simulink model "test_semiconductors_bridges"  (R2026b)
settings: Solver=ode23tb  StopTime=tb.t_stop
undefined symbols (not defined in the file or in its folder): tb
libraries: fl_lib x144, nesl_utility x54, single_phase_pwm_modulator x1, full_bridge_two_level_ideal_switch x1, full_bridge_two_level_igbt_simple_2th x1, full_bridge_two_level_mos_simple_2th x1, single_phase_three_levels_PWM_modulator x1, full_bridge_three_level_ttype_ideal_switch x1, full_bridge_three_level_ttype_igbt_simple_2th x1, full_bridge_three_level_ttype_mos_simple_2th x1, half_bridge_three_level_ttype_ideal_switch x1, half_bridge_three_level_ttype_igbt_simple_2th x1
(part 2 of 3)

== system test_semiconductors_bridges/modulator_1ph3L/test_half_bridge_three_level_ttype_mos_simple_2th ==
  gate_commands : Inport
  Electrical Reference : fl_lib/Electrical/Electrical Elements/Electrical Reference
  L : fl_lib/Electrical/Electrical Elements/Inductor  l=tb.load.L H  r=0 Ohm  g=0 1/Ohm  i_specify=off  i_priority=None  i=0 A  i_nominal_specify=off  i_nominal_value=1  i_nominal_unit=A  v_specify=off  v_priority=None  v=0 V  v_nominal_specify=off  v_nominal_value=1  v_nominal_unit=V  i_L_specify=off  i_L_priority=High  i_L=0 A  i_L_nominal_specify=off  i_L_nominal_value=1  i_L_nominal_unit=A
  R : fl_lib/Electrical/Electrical Elements/Resistor  R=tb.load.R Ohm  i_specify=off  i_priority=None  i=0 A  i_nominal_specify=off  i_nominal_value=1  i_nominal_unit=A  v_specify=off  v_priority=None  v=0 V  v_nominal_specify=off  v_nominal_value=1  v_nominal_unit=V
  Solver Configuration : nesl_utility/Solver Configuration  PhysicalDomain=network_engine_domain  SubClassName=solver  LeftPortType=input  RightPortType=generic  Tones=[]  Harmonics=[]  SimulateNoise=off  Profile=off  UseLocalSampling=off  EnableSwitchedLinearOptims=on  FrequencyDomain=off  UseCCode=off  RelTol=0.001  AbsTol=0.001  MinStep=1e-09  ToWorkspace=off  RevertToSquareIcSolve=off  NumHomotopyIterations=100  PhasorMode=off  PhasorModeNumHarmonics=1  ConsistencySolver=NEWTON_FTOL  CanonicalOrdering=UNORDERED  OptimizeIntermediates=UNOPTIMIZED  MulticoreSolverChoice=BACKWARD_EULER  IndexReductionMethod=DerivativeReplacement  DoDC=off  ResidualTolerance=1e-4  ConsistencyTolSource=GLOBAL  ConsistencyAbsTol=0.001  ConsistencyRelTol=0.001  ConsistencyTolFactor=0.001  UseLocalSolver=on  LocalSolverChoice=NE_BACKWARD_EULER_ADVANCER  ResolveIndetEquations=on  FunctionEvalNumThread=1  LocalSolverSampleTime=tb.tc  DoFixedCost=on  MaxNonlinIter=tb.nonlin_iter_ttype  MaxModeIter=tb.mode_iter  ComputeImpulses=off  ImpulseIterations=2  LinearAlgebra=auto  LinearAlgebraNumThread=0  EquationFormulation=NE_TIME_EF  DelaysMemoryBudget=1024  AutomaticFiltering=on  FilteringTimeConstant=0.001  PartitionStorageMethod=AS_NEEDED  PartitionMemoryBudget=1024  PartitionMethod=BALANCED  MultibodyUseLocalSolver=off  MultibodyLocalSolverChoice=ODE1  MultibodyLocalSolverSampleTime=0.001
  Vdc1 : fl_lib/Electrical/Electrical Sources/DC Voltage Source  v0=tb.Vdc/2 V
  Vdc2 : fl_lib/Electrical/Electrical Sources/DC Voltage Source  v0=tb.Vdc/2 V
  half_bridge_three_level_ttype_mos_simple_2th : half_bridge_three_level_ttype_mos_simple_2th/half_bridge_three_level_ttype_mos_simple_2th  rds_on_m=tb.mos.rds_on  alpha_R_m=tb.mos.alpha_R  Tj_ref_m=tb.mos.Tj_ref  Roff_m=tb.mos.Roff  v_gamma_m=tb.mos.v_gamma  rd_on_m=tb.mos.rd_on  two_die_m=tb.mos.two_die  G_th_m=tb.mos.G_th  Eon_m=tb.mos.Eon  Eoff_m=tb.mos.Eoff  Err_m=tb.mos.Err  Ic_ref_m=tb.mos.Ic_ref  Vdc_ref_m=tb.mos.Vdc_ref  ki_m=tb.mos.ki  kv_m=tb.mos.kv  Vth_off_m=tb.mos.Vth_off  Vth_on_m=tb.mos.Vth_on  V_sm_m=tb.mos.V_sm  time_constant_edge_m=tb.mos.time_constant_edge  tau_v_m=tb.mos.tau_v  time_constant_ploss_m=tb.mos.time_constant_ploss  i_eps_m=tb.mos.i_eps  Csnubber_m=tb.mos.Csnubber  Rsnubber_m=tb.mos.Rsnubber  rth_switch_JH_m=tb.mos.rth_switch_JH  rth_switch_HA_m=tb.mos.rth_switch_HA  rth_diode_JH_m=tb.mos.rth_diode_JH  rth_diode_HA_m=tb.mos.rth_diode_HA  JunctionTermalMass_m=tb.mos.JunctionTermalMass  Tambient_m=tb.mos.Tambient  mass_heatsink_m=tb.mos.mass_heatsink  specific_heat_m=tb.mos.specific_heat
  half_bridge_three_level_ttype_mos_simple_2th_i : ToWorkspace  VariableName=half_bridge_three_level_ttype_mos_simple_2th_i  SaveFormat=Timeseries  SampleTime=tb.ts_log
  half_bridge_three_level_ttype_mos_simple_2th_m : ToWorkspace  VariableName=half_bridge_three_level_ttype_mos_simple_2th_m  SaveFormat=Timeseries  SampleTime=tb.ts_log
  half_bridge_three_level_ttype_mos_simple_2th_u : ToWorkspace  VariableName=half_bridge_three_level_ttype_mos_simple_2th_u  SaveFormat=Timeseries  SampleTime=tb.ts_log
  i_A : nesl_utility/PS-Simulink Converter  PhysicalDomain=network_engine_domain  SubClassName=ps_output  LeftPortType=input  RightPortType=output  PseudoPeriodic=off  Frequencies=[]  VectorFormat=1-D array  Unit=A  AffineConversion=off
  i_load : fl_lib/Electrical/Electrical Sensors/Current Sensor
  u_V : nesl_utility/PS-Simulink Converter  PhysicalDomain=network_engine_domain  SubClassName=ps_output  LeftPortType=input  RightPortType=output  PseudoPeriodic=off  Frequencies=[]  VectorFormat=1-D array  Unit=V  AffineConversion=off
  u_load : fl_lib/Electrical/Electrical Sensors/Voltage Sensor
  wires:
  gate_commands/1 -> half_bridge_three_level_ttype_mos_simple_2th/1
  half_bridge_three_level_ttype_mos_simple_2th/1 -> half_bridge_three_level_ttype_mos_simple_2th_m/1
  i_A/1 -> half_bridge_three_level_ttype_mos_simple_2th_i/1
  u_V/1 -> half_bridge_three_level_ttype_mos_simple_2th_u/1
  connections:
  Vdc1/LConn1 -- half_bridge_three_level_ttype_mos_simple_2th/LConn1
  Vdc2/RConn1 -- half_bridge_three_level_ttype_mos_simple_2th/LConn3
  i_load/RConn1 -- i_A/LConn1
  u_load/RConn1 -- u_V/LConn1
  half_bridge_three_level_ttype_mos_simple_2th/RConn1 -- i_load/LConn1 -- u_load/LConn1
  i_load/RConn2 -- R/LConn1
  R/RConn1 -- L/LConn1
  L/RConn1 -- u_load/RConn2 -- Vdc1/RConn1 -- Vdc2/LConn1 -- Electrical Reference/LConn1 -- Solver Configuration/RConn1 -- half_bridge_three_level_ttype_mos_simple_2th/LConn2

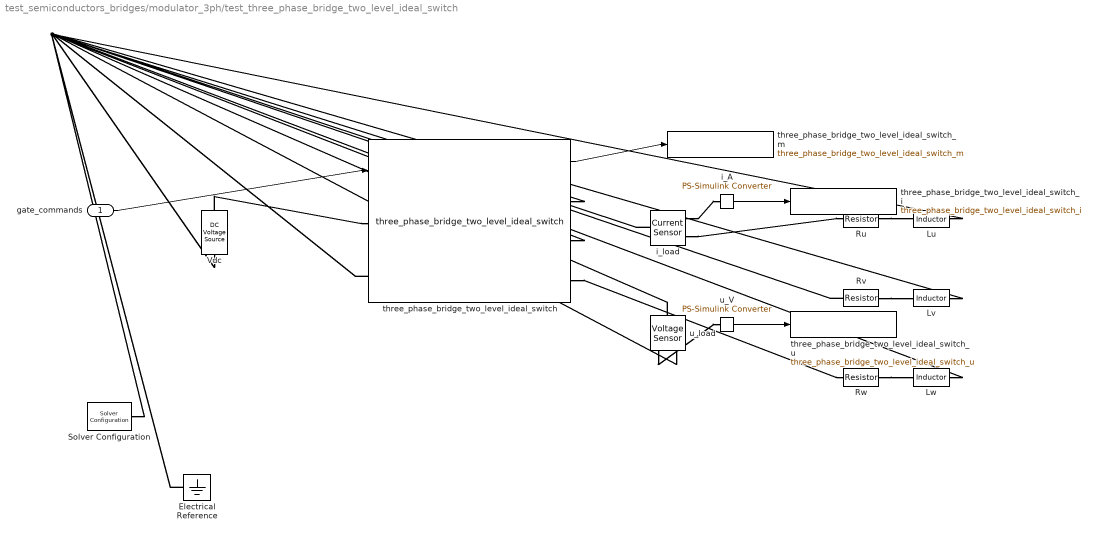
== system test_semiconductors_bridges/modulator_3ph/test_three_phase_bridge_two_level_ideal_switch ==
  gate_commands : Inport
  Electrical Reference : fl_lib/Electrical/Electrical Elements/Electrical Reference
  Lu : fl_lib/Electrical/Electrical Elements/Inductor  l=tb.load.L H  r=0 Ohm  g=0 1/Ohm  i_specify=off  i_priority=None  i=0 A  i_nominal_specify=off  i_nominal_value=1  i_nominal_unit=A  v_specify=off  v_priority=None  v=0 V  v_nominal_specify=off  v_nominal_value=1  v_nominal_unit=V  i_L_specify=off  i_L_priority=High  i_L=0 A  i_L_nominal_specify=off  i_L_nominal_value=1  i_L_nominal_unit=A
  Lv : fl_lib/Electrical/Electrical Elements/Inductor  l=tb.load.L H  r=0 Ohm  g=0 1/Ohm  i_specify=off  i_priority=None  i=0 A  i_nominal_specify=off  i_nominal_value=1  i_nominal_unit=A  v_specify=off  v_priority=None  v=0 V  v_nominal_specify=off  v_nominal_value=1  v_nominal_unit=V  i_L_specify=off  i_L_priority=High  i_L=0 A  i_L_nominal_specify=off  i_L_nominal_value=1  i_L_nominal_unit=A
  Lw : fl_lib/Electrical/Electrical Elements/Inductor  l=tb.load.L H  r=0 Ohm  g=0 1/Ohm  i_specify=off  i_priority=None  i=0 A  i_nominal_specify=off  i_nominal_value=1  i_nominal_unit=A  v_specify=off  v_priority=None  v=0 V  v_nominal_specify=off  v_nominal_value=1  v_nominal_unit=V  i_L_specify=off  i_L_priority=High  i_L=0 A  i_L_nominal_specify=off  i_L_nominal_value=1  i_L_nominal_unit=A
  Ru : fl_lib/Electrical/Electrical Elements/Resistor  R=tb.load.R Ohm  i_specify=off  i_priority=None  i=0 A  i_nominal_specify=off  i_nominal_value=1  i_nominal_unit=A  v_specify=off  v_priority=None  v=0 V  v_nominal_specify=off  v_nominal_value=1  v_nominal_unit=V
  Rv : fl_lib/Electrical/Electrical Elements/Resistor  R=tb.load.R Ohm  i_specify=off  i_priority=None  i=0 A  i_nominal_specify=off  i_nominal_value=1  i_nominal_unit=A  v_specify=off  v_priority=None  v=0 V  v_nominal_specify=off  v_nominal_value=1  v_nominal_unit=V
  Rw : fl_lib/Electrical/Electrical Elements/Resistor  R=tb.load.R Ohm  i_specify=off  i_priority=None  i=0 A  i_nominal_specify=off  i_nominal_value=1  i_nominal_unit=A  v_specify=off  v_priority=None  v=0 V  v_nominal_specify=off  v_nominal_value=1  v_nominal_unit=V
  Solver Configuration : nesl_utility/Solver Configuration  PhysicalDomain=network_engine_domain  SubClassName=solver  LeftPortType=input  RightPortType=generic  Tones=[]  Harmonics=[]  SimulateNoise=off  Profile=off  UseLocalSampling=off  EnableSwitchedLinearOptims=on  FrequencyDomain=off  UseCCode=off  RelTol=0.001  AbsTol=0.001  MinStep=1e-09  ToWorkspace=off  RevertToSquareIcSolve=off  NumHomotopyIterations=100  PhasorMode=off  PhasorModeNumHarmonics=1  ConsistencySolver=NEWTON_FTOL  CanonicalOrdering=UNORDERED  OptimizeIntermediates=UNOPTIMIZED  MulticoreSolverChoice=BACKWARD_EULER  IndexReductionMethod=DerivativeReplacement  DoDC=off  ResidualTolerance=1e-4  ConsistencyTolSource=GLOBAL  ConsistencyAbsTol=0.001  ConsistencyRelTol=0.001  ConsistencyTolFactor=0.001  UseLocalSolver=on  LocalSolverChoice=NE_BACKWARD_EULER_ADVANCER  ResolveIndetEquations=on  FunctionEvalNumThread=1  LocalSolverSampleTime=tb.tc  DoFixedCost=on  MaxNonlinIter=tb.nonlin_iter  MaxModeIter=tb.mode_iter  ComputeImpulses=off  ImpulseIterations=2  LinearAlgebra=auto  LinearAlgebraNumThread=0  EquationFormulation=NE_TIME_EF  DelaysMemoryBudget=1024  AutomaticFiltering=on  FilteringTimeConstant=0.001  PartitionStorageMethod=AS_NEEDED  PartitionMemoryBudget=1024  PartitionMethod=BALANCED  MultibodyUseLocalSolver=off  MultibodyLocalSolverChoice=ODE1  MultibodyLocalSolverSampleTime=0.001
  Vdc : fl_lib/Electrical/Electrical Sources/DC Voltage Source  v0=tb.Vdc V
  i_A : nesl_utility/PS-Simulink Converter  PhysicalDomain=network_engine_domain  SubClassName=ps_output  LeftPortType=input  RightPortType=output  PseudoPeriodic=off  Frequencies=[]  VectorFormat=1-D array  Unit=A  AffineConversion=off
  i_load : fl_lib/Electrical/Electrical Sensors/Current Sensor
  three_phase_bridge_two_level_ideal_switch : three_phase_bridge_two_level_ideal_switch/three_phase_bridge_two_level_ideal_switch  Rds_on=tb.ideal.Rds_on  Vdon_diode=tb.ideal.Vdon_diode  Rdon_diode=tb.ideal.Rdon_diode  Csnubber=tb.ideal.Csnubber  Rsnubber=tb.ideal.Rsnubber  Vth=tb.ideal.Vth
  three_phase_bridge_two_level_ideal_switch_i : ToWorkspace  VariableName=three_phase_bridge_two_level_ideal_switch_i  SaveFormat=Timeseries  SampleTime=tb.ts_log
  three_phase_bridge_two_level_ideal_switch_m : ToWorkspace  VariableName=three_phase_bridge_two_level_ideal_switch_m  SaveFormat=Timeseries  SampleTime=tb.ts_log
  three_phase_bridge_two_level_ideal_switch_u : ToWorkspace  VariableName=three_phase_bridge_two_level_ideal_switch_u  SaveFormat=Timeseries  SampleTime=tb.ts_log
  u_V : nesl_utility/PS-Simulink Converter  PhysicalDomain=network_engine_domain  SubClassName=ps_output  LeftPortType=input  RightPortType=output  PseudoPeriodic=off  Frequencies=[]  VectorFormat=1-D array  Unit=V  AffineConversion=off
  u_load : fl_lib/Electrical/Electrical Sensors/Voltage Sensor
  wires:
  gate_commands/1 -> three_phase_bridge_two_level_ideal_switch/1
  three_phase_bridge_two_level_ideal_switch/1 -> three_phase_bridge_two_level_ideal_switch_m/1
  i_A/1 -> three_phase_bridge_two_level_ideal_switch_i/1
  u_V/1 -> three_phase_bridge_two_level_ideal_switch_u/1
  connections:
  Vdc/LConn1 -- three_phase_bridge_two_level_ideal_switch/LConn1
  Vdc/RConn1 -- three_phase_bridge_two_level_ideal_switch/LConn2 -- Electrical Reference/LConn1 -- Solver Configuration/RConn1
  i_load/RConn1 -- i_A/LConn1
  u_load/RConn1 -- u_V/LConn1
  i_load/RConn2 -- Ru/LConn1
  Ru/RConn1 -- Lu/LConn1
  three_phase_bridge_two_level_ideal_switch/RConn2 -- Rv/LConn1 -- u_load/RConn2
  Rv/RConn1 -- Lv/LConn1
  three_phase_bridge_two_level_ideal_switch/RConn3 -- Rw/LConn1
  Rw/RConn1 -- Lw/LConn1
  Lu/RConn1 -- Lv/RConn1 -- Lw/RConn1
  three_phase_bridge_two_level_ideal_switch/RConn1 -- i_load/LConn1 -- u_load/LConn1

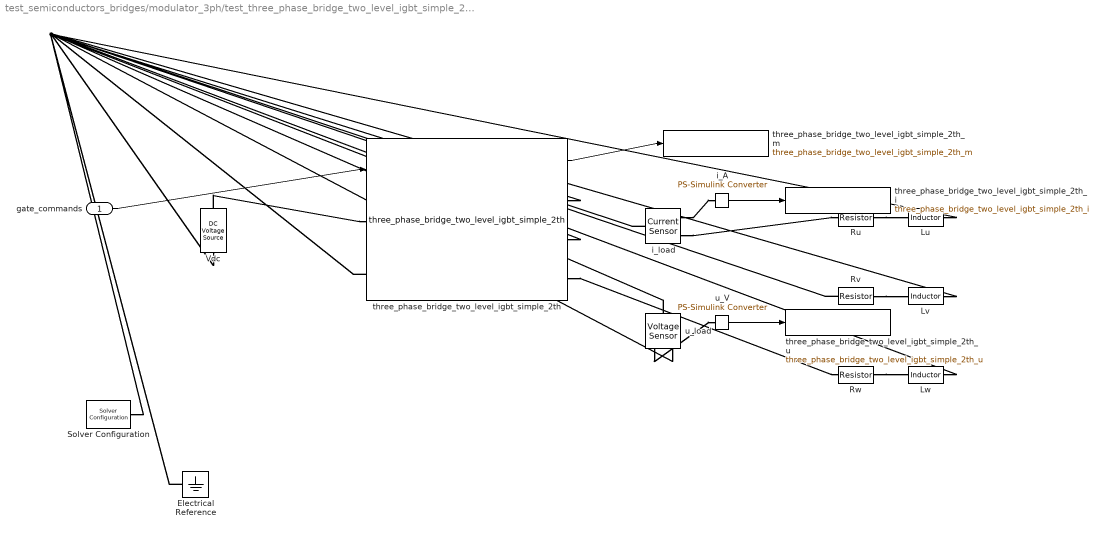
== system test_semiconductors_bridges/modulator_3ph/test_three_phase_bridge_two_level_igbt_simple_2th ==
  gate_commands : Inport
  Electrical Reference : fl_lib/Electrical/Electrical Elements/Electrical Reference
  Lu : fl_lib/Electrical/Electrical Elements/Inductor  l=tb.load.L H  r=0 Ohm  g=0 1/Ohm  i_specify=off  i_priority=None  i=0 A  i_nominal_specify=off  i_nominal_value=1  i_nominal_unit=A  v_specify=off  v_priority=None  v=0 V  v_nominal_specify=off  v_nominal_value=1  v_nominal_unit=V  i_L_specify=off  i_L_priority=High  i_L=0 A  i_L_nominal_specify=off  i_L_nominal_value=1  i_L_nominal_unit=A
  Lv : fl_lib/Electrical/Electrical Elements/Inductor  l=tb.load.L H  r=0 Ohm  g=0 1/Ohm  i_specify=off  i_priority=None  i=0 A  i_nominal_specify=off  i_nominal_value=1  i_nominal_unit=A  v_specify=off  v_priority=None  v=0 V  v_nominal_specify=off  v_nominal_value=1  v_nominal_unit=V  i_L_specify=off  i_L_priority=High  i_L=0 A  i_L_nominal_specify=off  i_L_nominal_value=1  i_L_nominal_unit=A
  Lw : fl_lib/Electrical/Electrical Elements/Inductor  l=tb.load.L H  r=0 Ohm  g=0 1/Ohm  i_specify=off  i_priority=None  i=0 A  i_nominal_specify=off  i_nominal_value=1  i_nominal_unit=A  v_specify=off  v_priority=None  v=0 V  v_nominal_specify=off  v_nominal_value=1  v_nominal_unit=V  i_L_specify=off  i_L_priority=High  i_L=0 A  i_L_nominal_specify=off  i_L_nominal_value=1  i_L_nominal_unit=A
  Ru : fl_lib/Electrical/Electrical Elements/Resistor  R=tb.load.R Ohm  i_specify=off  i_priority=None  i=0 A  i_nominal_specify=off  i_nominal_value=1  i_nominal_unit=A  v_specify=off  v_priority=None  v=0 V  v_nominal_specify=off  v_nominal_value=1  v_nominal_unit=V
  Rv : fl_lib/Electrical/Electrical Elements/Resistor  R=tb.load.R Ohm  i_specify=off  i_priority=None  i=0 A  i_nominal_specify=off  i_nominal_value=1  i_nominal_unit=A  v_specify=off  v_priority=None  v=0 V  v_nominal_specify=off  v_nominal_value=1  v_nominal_unit=V
  Rw : fl_lib/Electrical/Electrical Elements/Resistor  R=tb.load.R Ohm  i_specify=off  i_priority=None  i=0 A  i_nominal_specify=off  i_nominal_value=1  i_nominal_unit=A  v_specify=off  v_priority=None  v=0 V  v_nominal_specify=off  v_nominal_value=1  v_nominal_unit=V
  Solver Configuration : nesl_utility/Solver Configuration  PhysicalDomain=network_engine_domain  SubClassName=solver  LeftPortType=input  RightPortType=generic  Tones=[]  Harmonics=[]  SimulateNoise=off  Profile=off  UseLocalSampling=off  EnableSwitchedLinearOptims=on  FrequencyDomain=off  UseCCode=off  RelTol=0.001  AbsTol=0.001  MinStep=1e-09  ToWorkspace=off  RevertToSquareIcSolve=off  NumHomotopyIterations=100  PhasorMode=off  PhasorModeNumHarmonics=1  ConsistencySolver=NEWTON_FTOL  CanonicalOrdering=UNORDERED  OptimizeIntermediates=UNOPTIMIZED  MulticoreSolverChoice=BACKWARD_EULER  IndexReductionMethod=DerivativeReplacement  DoDC=off  ResidualTolerance=1e-4  ConsistencyTolSource=GLOBAL  ConsistencyAbsTol=0.001  ConsistencyRelTol=0.001  ConsistencyTolFactor=0.001  UseLocalSolver=on  LocalSolverChoice=NE_BACKWARD_EULER_ADVANCER  ResolveIndetEquations=on  FunctionEvalNumThread=1  LocalSolverSampleTime=tb.tc  DoFixedCost=on  MaxNonlinIter=tb.nonlin_iter  MaxModeIter=tb.mode_iter  ComputeImpulses=off  ImpulseIterations=2  LinearAlgebra=auto  LinearAlgebraNumThread=0  EquationFormulation=NE_TIME_EF  DelaysMemoryBudget=1024  AutomaticFiltering=on  FilteringTimeConstant=0.001  PartitionStorageMethod=AS_NEEDED  PartitionMemoryBudget=1024  PartitionMethod=BALANCED  MultibodyUseLocalSolver=off  MultibodyLocalSolverChoice=ODE1  MultibodyLocalSolverSampleTime=0.001
  Vdc : fl_lib/Electrical/Electrical Sources/DC Voltage Source  v0=tb.Vdc V
  i_A : nesl_utility/PS-Simulink Converter  PhysicalDomain=network_engine_domain  SubClassName=ps_output  LeftPortType=input  RightPortType=output  PseudoPeriodic=off  Frequencies=[]  VectorFormat=1-D array  Unit=A  AffineConversion=off
  i_load : fl_lib/Electrical/Electrical Sensors/Current Sensor
  three_phase_bridge_two_level_igbt_simple_2th : three_phase_bridge_two_level_igbt_simple_2th/three_phase_bridge_two_level_igbt_simple_2th  vce_sat_m=tb.igbt.vce_sat  rce_on_m=tb.igbt.rce_on  v_gamma_m=tb.igbt.v_gamma  rd_on_m=tb.igbt.rd_on  Gce_off_m=tb.igbt.Gce_off  Vth_gate_m=tb.igbt.Vth_gate  Vth_gate_hyst_m=tb.igbt.Vth_gate_hyst  Eon_m=tb.igbt.Eon  Eoff_m=tb.igbt.Eoff  Err_m=tb.igbt.Err  Ic_ref_m=tb.igbt.Ic_ref  Vdc_ref_m=tb.igbt.Vdc_ref  Vblock_Errf_m=tb.igbt.Vblock_Errf  time_constant_edge_m=tb.igbt.time_constant_edge  time_constant_ploss_m=tb.igbt.time_constant_ploss  Csnubber_m=tb.igbt.Csnubber  Rsnubber_m=tb.igbt.Rsnubber  rth_switch_JH_m=tb.igbt.rth_switch_JH  rth_switch_HA_m=tb.igbt.rth_switch_HA  rth_diode_JH_m=tb.igbt.rth_diode_JH  rth_diode_HA_m=tb.igbt.rth_diode_HA  JunctionTermalMass_m=tb.igbt.JunctionTermalMass  Tambient_m=tb.igbt.Tambient  mass_heatsink_m=tb.igbt.mass_heatsink  specific_heat_m=tb.igbt.specific_heat
  three_phase_bridge_two_level_igbt_simple_2th_i : ToWorkspace  VariableName=three_phase_bridge_two_level_igbt_simple_2th_i  SaveFormat=Timeseries  SampleTime=tb.ts_log
  three_phase_bridge_two_level_igbt_simple_2th_m : ToWorkspace  VariableName=three_phase_bridge_two_level_igbt_simple_2th_m  SaveFormat=Timeseries  SampleTime=tb.ts_log
  three_phase_bridge_two_level_igbt_simple_2th_u : ToWorkspace  VariableName=three_phase_bridge_two_level_igbt_simple_2th_u  SaveFormat=Timeseries  SampleTime=tb.ts_log
  u_V : nesl_utility/PS-Simulink Converter  PhysicalDomain=network_engine_domain  SubClassName=ps_output  LeftPortType=input  RightPortType=output  PseudoPeriodic=off  Frequencies=[]  VectorFormat=1-D array  Unit=V  AffineConversion=off
  u_load : fl_lib/Electrical/Electrical Sensors/Voltage Sensor
  wires:
  gate_commands/1 -> three_phase_bridge_two_level_igbt_simple_2th/1
  three_phase_bridge_two_level_igbt_simple_2th/1 -> three_phase_bridge_two_level_igbt_simple_2th_m/1
  i_A/1 -> three_phase_bridge_two_level_igbt_simple_2th_i/1
  u_V/1 -> three_phase_bridge_two_level_igbt_simple_2th_u/1
  connections:
  Vdc/LConn1 -- three_phase_bridge_two_level_igbt_simple_2th/LConn1
  Vdc/RConn1 -- three_phase_bridge_two_level_igbt_simple_2th/LConn2 -- Electrical Reference/LConn1 -- Solver Configuration/RConn1
  i_load/RConn1 -- i_A/LConn1
  u_load/RConn1 -- u_V/LConn1
  i_load/RConn2 -- Ru/LConn1
  Ru/RConn1 -- Lu/LConn1
  three_phase_bridge_two_level_igbt_simple_2th/RConn2 -- Rv/LConn1 -- u_load/RConn2
  Rv/RConn1 -- Lv/LConn1
  three_phase_bridge_two_level_igbt_simple_2th/RConn3 -- Rw/LConn1
  Rw/RConn1 -- Lw/LConn1
  Lu/RConn1 -- Lv/RConn1 -- Lw/RConn1
  three_phase_bridge_two_level_igbt_simple_2th/RConn1 -- i_load/LConn1 -- u_load/LConn1

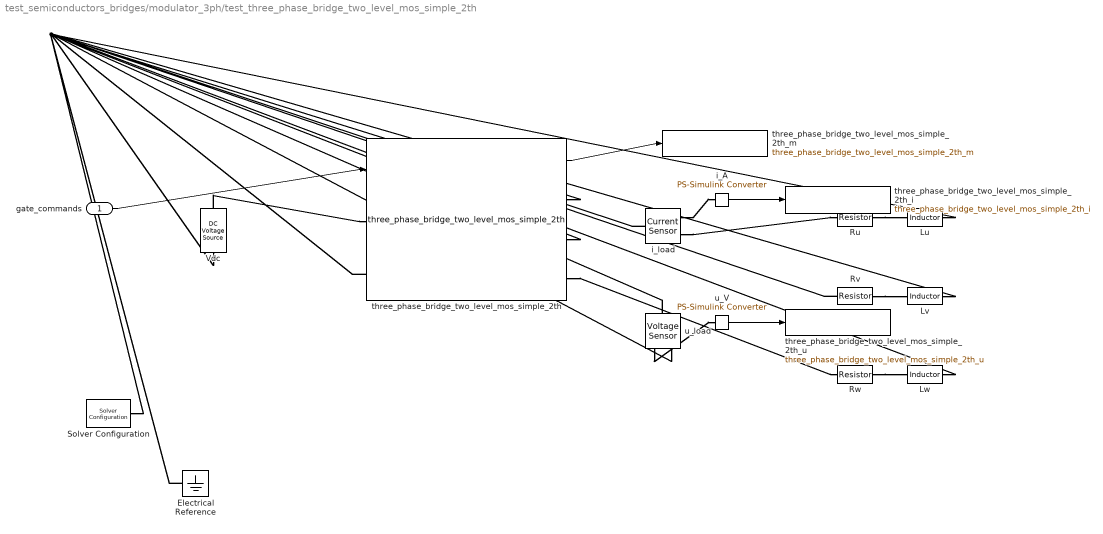
== system test_semiconductors_bridges/modulator_3ph/test_three_phase_bridge_two_level_mos_simple_2th ==
  gate_commands : Inport
  Electrical Reference : fl_lib/Electrical/Electrical Elements/Electrical Reference
  Lu : fl_lib/Electrical/Electrical Elements/Inductor  l=tb.load.L H  r=0 Ohm  g=0 1/Ohm  i_specify=off  i_priority=None  i=0 A  i_nominal_specify=off  i_nominal_value=1  i_nominal_unit=A  v_specify=off  v_priority=None  v=0 V  v_nominal_specify=off  v_nominal_value=1  v_nominal_unit=V  i_L_specify=off  i_L_priority=High  i_L=0 A  i_L_nominal_specify=off  i_L_nominal_value=1  i_L_nominal_unit=A
  Lv : fl_lib/Electrical/Electrical Elements/Inductor  l=tb.load.L H  r=0 Ohm  g=0 1/Ohm  i_specify=off  i_priority=None  i=0 A  i_nominal_specify=off  i_nominal_value=1  i_nominal_unit=A  v_specify=off  v_priority=None  v=0 V  v_nominal_specify=off  v_nominal_value=1  v_nominal_unit=V  i_L_specify=off  i_L_priority=High  i_L=0 A  i_L_nominal_specify=off  i_L_nominal_value=1  i_L_nominal_unit=A
  Lw : fl_lib/Electrical/Electrical Elements/Inductor  l=tb.load.L H  r=0 Ohm  g=0 1/Ohm  i_specify=off  i_priority=None  i=0 A  i_nominal_specify=off  i_nominal_value=1  i_nominal_unit=A  v_specify=off  v_priority=None  v=0 V  v_nominal_specify=off  v_nominal_value=1  v_nominal_unit=V  i_L_specify=off  i_L_priority=High  i_L=0 A  i_L_nominal_specify=off  i_L_nominal_value=1  i_L_nominal_unit=A
  Ru : fl_lib/Electrical/Electrical Elements/Resistor  R=tb.load.R Ohm  i_specify=off  i_priority=None  i=0 A  i_nominal_specify=off  i_nominal_value=1  i_nominal_unit=A  v_specify=off  v_priority=None  v=0 V  v_nominal_specify=off  v_nominal_value=1  v_nominal_unit=V
  Rv : fl_lib/Electrical/Electrical Elements/Resistor  R=tb.load.R Ohm  i_specify=off  i_priority=None  i=0 A  i_nominal_specify=off  i_nominal_value=1  i_nominal_unit=A  v_specify=off  v_priority=None  v=0 V  v_nominal_specify=off  v_nominal_value=1  v_nominal_unit=V
  Rw : fl_lib/Electrical/Electrical Elements/Resistor  R=tb.load.R Ohm  i_specify=off  i_priority=None  i=0 A  i_nominal_specify=off  i_nominal_value=1  i_nominal_unit=A  v_specify=off  v_priority=None  v=0 V  v_nominal_specify=off  v_nominal_value=1  v_nominal_unit=V
  Solver Configuration : nesl_utility/Solver Configuration  PhysicalDomain=network_engine_domain  SubClassName=solver  LeftPortType=input  RightPortType=generic  Tones=[]  Harmonics=[]  SimulateNoise=off  Profile=off  UseLocalSampling=off  EnableSwitchedLinearOptims=on  FrequencyDomain=off  UseCCode=off  RelTol=0.001  AbsTol=0.001  MinStep=1e-09  ToWorkspace=off  RevertToSquareIcSolve=off  NumHomotopyIterations=100  PhasorMode=off  PhasorModeNumHarmonics=1  ConsistencySolver=NEWTON_FTOL  CanonicalOrdering=UNORDERED  OptimizeIntermediates=UNOPTIMIZED  MulticoreSolverChoice=BACKWARD_EULER  IndexReductionMethod=DerivativeReplacement  DoDC=off  ResidualTolerance=1e-4  ConsistencyTolSource=GLOBAL  ConsistencyAbsTol=0.001  ConsistencyRelTol=0.001  ConsistencyTolFactor=0.001  UseLocalSolver=on  LocalSolverChoice=NE_BACKWARD_EULER_ADVANCER  ResolveIndetEquations=on  FunctionEvalNumThread=1  LocalSolverSampleTime=tb.tc  DoFixedCost=on  MaxNonlinIter=tb.nonlin_iter  MaxModeIter=tb.mode_iter  ComputeImpulses=off  ImpulseIterations=2  LinearAlgebra=auto  LinearAlgebraNumThread=0  EquationFormulation=NE_TIME_EF  DelaysMemoryBudget=1024  AutomaticFiltering=on  FilteringTimeConstant=0.001  PartitionStorageMethod=AS_NEEDED  PartitionMemoryBudget=1024  PartitionMethod=BALANCED  MultibodyUseLocalSolver=off  MultibodyLocalSolverChoice=ODE1  MultibodyLocalSolverSampleTime=0.001
  Vdc : fl_lib/Electrical/Electrical Sources/DC Voltage Source  v0=tb.Vdc V
  i_A : nesl_utility/PS-Simulink Converter  PhysicalDomain=network_engine_domain  SubClassName=ps_output  LeftPortType=input  RightPortType=output  PseudoPeriodic=off  Frequencies=[]  VectorFormat=1-D array  Unit=A  AffineConversion=off
  i_load : fl_lib/Electrical/Electrical Sensors/Current Sensor
  three_phase_bridge_two_level_mos_simple_2th : three_phase_bridge_two_level_mos_simple_2th/three_phase_bridge_two_level_mos_simple_2th  rds_on_m=tb.mos.rds_on  alpha_R_m=tb.mos.alpha_R  Tj_ref_m=tb.mos.Tj_ref  Roff_m=tb.mos.Roff  v_gamma_m=tb.mos.v_gamma  rd_on_m=tb.mos.rd_on  two_die_m=tb.mos.two_die  G_th_m=tb.mos.G_th  Eon_m=tb.mos.Eon  Eoff_m=tb.mos.Eoff  Err_m=tb.mos.Err  Ic_ref_m=tb.mos.Ic_ref  Vdc_ref_m=tb.mos.Vdc_ref  ki_m=tb.mos.ki  kv_m=tb.mos.kv  Vth_off_m=tb.mos.Vth_off  Vth_on_m=tb.mos.Vth_on  V_sm_m=tb.mos.V_sm  time_constant_edge_m=tb.mos.time_constant_edge  tau_v_m=tb.mos.tau_v  time_constant_ploss_m=tb.mos.time_constant_ploss  i_eps_m=tb.mos.i_eps  Csnubber_m=tb.mos.Csnubber  Rsnubber_m=tb.mos.Rsnubber  rth_switch_JH_m=tb.mos.rth_switch_JH  rth_switch_HA_m=tb.mos.rth_switch_HA  rth_diode_JH_m=tb.mos.rth_diode_JH  rth_diode_HA_m=tb.mos.rth_diode_HA  JunctionTermalMass_m=tb.mos.JunctionTermalMass  Tambient_m=tb.mos.Tambient  mass_heatsink_m=tb.mos.mass_heatsink  specific_heat_m=tb.mos.specific_heat
  three_phase_bridge_two_level_mos_simple_2th_i : ToWorkspace  VariableName=three_phase_bridge_two_level_mos_simple_2th_i  SaveFormat=Timeseries  SampleTime=tb.ts_log
  three_phase_bridge_two_level_mos_simple_2th_m : ToWorkspace  VariableName=three_phase_bridge_two_level_mos_simple_2th_m  SaveFormat=Timeseries  SampleTime=tb.ts_log
  three_phase_bridge_two_level_mos_simple_2th_u : ToWorkspace  VariableName=three_phase_bridge_two_level_mos_simple_2th_u  SaveFormat=Timeseries  SampleTime=tb.ts_log
  u_V : nesl_utility/PS-Simulink Converter  PhysicalDomain=network_engine_domain  SubClassName=ps_output  LeftPortType=input  RightPortType=output  PseudoPeriodic=off  Frequencies=[]  VectorFormat=1-D array  Unit=V  AffineConversion=off
  u_load : fl_lib/Electrical/Electrical Sensors/Voltage Sensor
  wires:
  gate_commands/1 -> three_phase_bridge_two_level_mos_simple_2th/1
  three_phase_bridge_two_level_mos_simple_2th/1 -> three_phase_bridge_two_level_mos_simple_2th_m/1
  i_A/1 -> three_phase_bridge_two_level_mos_simple_2th_i/1
  u_V/1 -> three_phase_bridge_two_level_mos_simple_2th_u/1
  connections:
  Vdc/LConn1 -- three_phase_bridge_two_level_mos_simple_2th/LConn1
  Vdc/RConn1 -- three_phase_bridge_two_level_mos_simple_2th/LConn2 -- Electrical Reference/LConn1 -- Solver Configuration/RConn1
  i_load/RConn1 -- i_A/LConn1
  u_load/RConn1 -- u_V/LConn1
  i_load/RConn2 -- Ru/LConn1
  Ru/RConn1 -- Lu/LConn1
  three_phase_bridge_two_level_mos_simple_2th/RConn2 -- Rv/LConn1 -- u_load/RConn2
  Rv/RConn1 -- Lv/LConn1
  three_phase_bridge_two_level_mos_simple_2th/RConn3 -- Rw/LConn1
  Rw/RConn1 -- Lw/LConn1
  Lu/RConn1 -- Lv/RConn1 -- Lw/RConn1
  three_phase_bridge_two_level_mos_simple_2th/RConn1 -- i_load/LConn1 -- u_load/LConn1

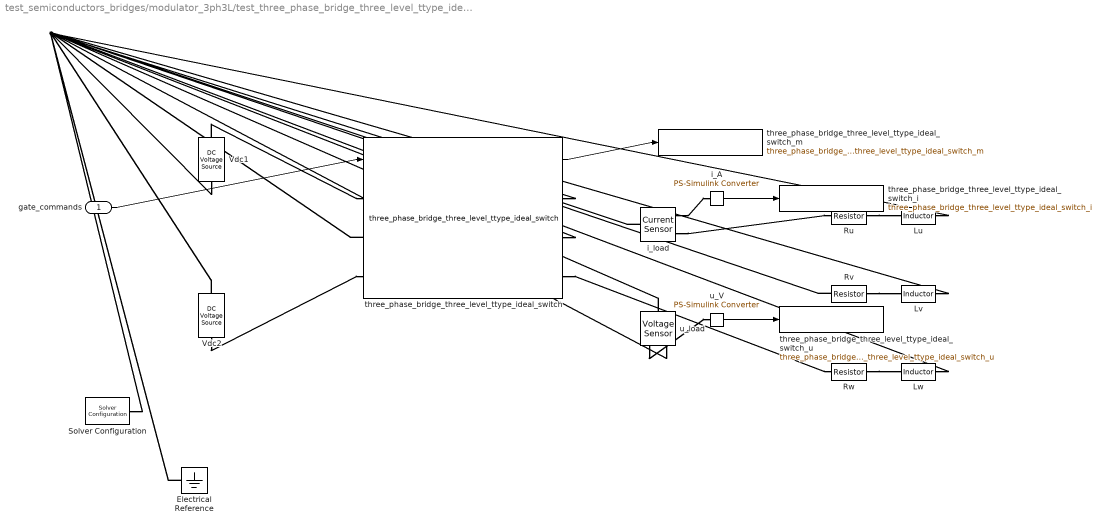
== system test_semiconductors_bridges/modulator_3ph3L/test_three_phase_bridge_three_level_ttype_ideal_switch ==
  gate_commands : Inport
  Electrical Reference : fl_lib/Electrical/Electrical Elements/Electrical Reference
  Lu : fl_lib/Electrical/Electrical Elements/Inductor  l=tb.load.L H  r=0 Ohm  g=0 1/Ohm  i_specify=off  i_priority=None  i=0 A  i_nominal_specify=off  i_nominal_value=1  i_nominal_unit=A  v_specify=off  v_priority=None  v=0 V  v_nominal_specify=off  v_nominal_value=1  v_nominal_unit=V  i_L_specify=off  i_L_priority=High  i_L=0 A  i_L_nominal_specify=off  i_L_nominal_value=1  i_L_nominal_unit=A
  Lv : fl_lib/Electrical/Electrical Elements/Inductor  l=tb.load.L H  r=0 Ohm  g=0 1/Ohm  i_specify=off  i_priority=None  i=0 A  i_nominal_specify=off  i_nominal_value=1  i_nominal_unit=A  v_specify=off  v_priority=None  v=0 V  v_nominal_specify=off  v_nominal_value=1  v_nominal_unit=V  i_L_specify=off  i_L_priority=High  i_L=0 A  i_L_nominal_specify=off  i_L_nominal_value=1  i_L_nominal_unit=A
  Lw : fl_lib/Electrical/Electrical Elements/Inductor  l=tb.load.L H  r=0 Ohm  g=0 1/Ohm  i_specify=off  i_priority=None  i=0 A  i_nominal_specify=off  i_nominal_value=1  i_nominal_unit=A  v_specify=off  v_priority=None  v=0 V  v_nominal_specify=off  v_nominal_value=1  v_nominal_unit=V  i_L_specify=off  i_L_priority=High  i_L=0 A  i_L_nominal_specify=off  i_L_nominal_value=1  i_L_nominal_unit=A
  Ru : fl_lib/Electrical/Electrical Elements/Resistor  R=tb.load.R Ohm  i_specify=off  i_priority=None  i=0 A  i_nominal_specify=off  i_nominal_value=1  i_nominal_unit=A  v_specify=off  v_priority=None  v=0 V  v_nominal_specify=off  v_nominal_value=1  v_nominal_unit=V
  Rv : fl_lib/Electrical/Electrical Elements/Resistor  R=tb.load.R Ohm  i_specify=off  i_priority=None  i=0 A  i_nominal_specify=off  i_nominal_value=1  i_nominal_unit=A  v_specify=off  v_priority=None  v=0 V  v_nominal_specify=off  v_nominal_value=1  v_nominal_unit=V
  Rw : fl_lib/Electrical/Electrical Elements/Resistor  R=tb.load.R Ohm  i_specify=off  i_priority=None  i=0 A  i_nominal_specify=off  i_nominal_value=1  i_nominal_unit=A  v_specify=off  v_priority=None  v=0 V  v_nominal_specify=off  v_nominal_value=1  v_nominal_unit=V
  Solver Configuration : nesl_utility/Solver Configuration  PhysicalDomain=network_engine_domain  SubClassName=solver  LeftPortType=input  RightPortType=generic  Tones=[]  Harmonics=[]  SimulateNoise=off  Profile=off  UseLocalSampling=off  EnableSwitchedLinearOptims=on  FrequencyDomain=off  UseCCode=off  RelTol=0.001  AbsTol=0.001  MinStep=1e-09  ToWorkspace=off  RevertToSquareIcSolve=off  NumHomotopyIterations=100  PhasorMode=off  PhasorModeNumHarmonics=1  ConsistencySolver=NEWTON_FTOL  CanonicalOrdering=UNORDERED  OptimizeIntermediates=UNOPTIMIZED  MulticoreSolverChoice=BACKWARD_EULER  IndexReductionMethod=DerivativeReplacement  DoDC=off  ResidualTolerance=1e-4  ConsistencyTolSource=GLOBAL  ConsistencyAbsTol=0.001  ConsistencyRelTol=0.001  ConsistencyTolFactor=0.001  UseLocalSolver=on  LocalSolverChoice=NE_BACKWARD_EULER_ADVANCER  ResolveIndetEquations=on  FunctionEvalNumThread=1  LocalSolverSampleTime=tb.tc  DoFixedCost=on  MaxNonlinIter=tb.nonlin_iter_ttype  MaxModeIter=tb.mode_iter  ComputeImpulses=off  ImpulseIterations=2  LinearAlgebra=auto  LinearAlgebraNumThread=0  EquationFormulation=NE_TIME_EF  DelaysMemoryBudget=1024  AutomaticFiltering=on  FilteringTimeConstant=0.001  PartitionStorageMethod=AS_NEEDED  PartitionMemoryBudget=1024  PartitionMethod=BALANCED  MultibodyUseLocalSolver=off  MultibodyLocalSolverChoice=ODE1  MultibodyLocalSolverSampleTime=0.001
  Vdc1 : fl_lib/Electrical/Electrical Sources/DC Voltage Source  v0=tb.Vdc/2 V
  Vdc2 : fl_lib/Electrical/Electrical Sources/DC Voltage Source  v0=tb.Vdc/2 V
  i_A : nesl_utility/PS-Simulink Converter  PhysicalDomain=network_engine_domain  SubClassName=ps_output  LeftPortType=input  RightPortType=output  PseudoPeriodic=off  Frequencies=[]  VectorFormat=1-D array  Unit=A  AffineConversion=off
  i_load : fl_lib/Electrical/Electrical Sensors/Current Sensor
  three_phase_bridge_three_level_ttype_ideal_switch : three_phase_bridge_three_level_ttype_ideal_switch/three_phase_bridge_three_level_ttype_ideal_switch  Rds_on=tb.ideal.Rds_on  Vdon_diode=tb.ideal.Vdon_diode  Rdon_diode=tb.ideal.Rdon_diode  Csnubber=tb.ideal.Csnubber  Rsnubber=tb.ideal.Rsnubber  Vth=tb.ideal.Vth
  three_phase_bridge_three_level_ttype_ideal_switch_i : ToWorkspace  VariableName=three_phase_bridge_three_level_ttype_ideal_switch_i  SaveFormat=Timeseries  SampleTime=tb.ts_log
  three_phase_bridge_three_level_ttype_ideal_switch_m : ToWorkspace  VariableName=three_phase_bridge_three_level_ttype_ideal_switch_m  SaveFormat=Timeseries  SampleTime=tb.ts_log
  three_phase_bridge_three_level_ttype_ideal_switch_u : ToWorkspace  VariableName=three_phase_bridge_three_level_ttype_ideal_switch_u  SaveFormat=Timeseries  SampleTime=tb.ts_log
  u_V : nesl_utility/PS-Simulink Converter  PhysicalDomain=network_engine_domain  SubClassName=ps_output  LeftPortType=input  RightPortType=output  PseudoPeriodic=off  Frequencies=[]  VectorFormat=1-D array  Unit=V  AffineConversion=off
  u_load : fl_lib/Electrical/Electrical Sensors/Voltage Sensor
  wires:
  gate_commands/1 -> three_phase_bridge_three_level_ttype_ideal_switch/1
  three_phase_bridge_three_level_ttype_ideal_switch/1 -> three_phase_bridge_three_level_ttype_ideal_switch_m/1
  i_A/1 -> three_phase_bridge_three_level_ttype_ideal_switch_i/1
  u_V/1 -> three_phase_bridge_three_level_ttype_ideal_switch_u/1
  connections:
  Vdc1/LConn1 -- three_phase_bridge_three_level_ttype_ideal_switch/LConn1
  Vdc2/RConn1 -- three_phase_bridge_three_level_ttype_ideal_switch/LConn3
  i_load/RConn1 -- i_A/LConn1
  u_load/RConn1 -- u_V/LConn1
  i_load/RConn2 -- Ru/LConn1
  Ru/RConn1 -- Lu/LConn1
  three_phase_bridge_three_level_ttype_ideal_switch/RConn2 -- Rv/LConn1 -- u_load/RConn2
  Rv/RConn1 -- Lv/LConn1
  three_phase_bridge_three_level_ttype_ideal_switch/RConn3 -- Rw/LConn1
  Rw/RConn1 -- Lw/LConn1
  Lu/RConn1 -- Lv/RConn1 -- Lw/RConn1
  three_phase_bridge_three_level_ttype_ideal_switch/RConn1 -- i_load/LConn1 -- u_load/LConn1
  Vdc1/RConn1 -- Vdc2/LConn1 -- Electrical Reference/LConn1 -- Solver Configuration/RConn1 -- three_phase_bridge_three_level_ttype_ideal_switch/LConn2

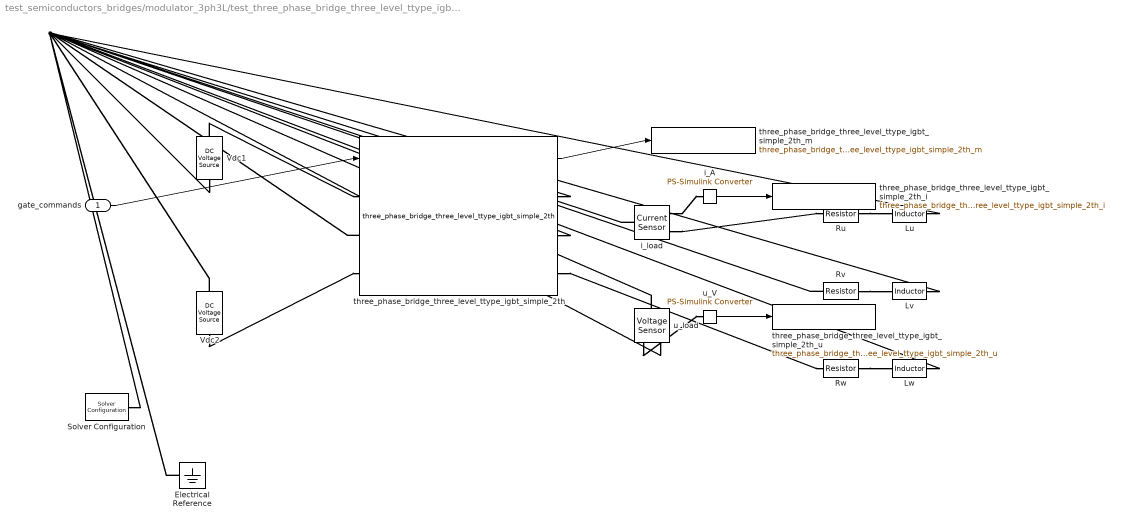
== system test_semiconductors_bridges/modulator_3ph3L/test_three_phase_bridge_three_level_ttype_igbt_simple_2th ==
  gate_commands : Inport
  Electrical Reference : fl_lib/Electrical/Electrical Elements/Electrical Reference
  Lu : fl_lib/Electrical/Electrical Elements/Inductor  l=tb.load.L H  r=0 Ohm  g=0 1/Ohm  i_specify=off  i_priority=None  i=0 A  i_nominal_specify=off  i_nominal_value=1  i_nominal_unit=A  v_specify=off  v_priority=None  v=0 V  v_nominal_specify=off  v_nominal_value=1  v_nominal_unit=V  i_L_specify=off  i_L_priority=High  i_L=0 A  i_L_nominal_specify=off  i_L_nominal_value=1  i_L_nominal_unit=A
  Lv : fl_lib/Electrical/Electrical Elements/Inductor  l=tb.load.L H  r=0 Ohm  g=0 1/Ohm  i_specify=off  i_priority=None  i=0 A  i_nominal_specify=off  i_nominal_value=1  i_nominal_unit=A  v_specify=off  v_priority=None  v=0 V  v_nominal_specify=off  v_nominal_value=1  v_nominal_unit=V  i_L_specify=off  i_L_priority=High  i_L=0 A  i_L_nominal_specify=off  i_L_nominal_value=1  i_L_nominal_unit=A
  Lw : fl_lib/Electrical/Electrical Elements/Inductor  l=tb.load.L H  r=0 Ohm  g=0 1/Ohm  i_specify=off  i_priority=None  i=0 A  i_nominal_specify=off  i_nominal_value=1  i_nominal_unit=A  v_specify=off  v_priority=None  v=0 V  v_nominal_specify=off  v_nominal_value=1  v_nominal_unit=V  i_L_specify=off  i_L_priority=High  i_L=0 A  i_L_nominal_specify=off  i_L_nominal_value=1  i_L_nominal_unit=A
  Ru : fl_lib/Electrical/Electrical Elements/Resistor  R=tb.load.R Ohm  i_specify=off  i_priority=None  i=0 A  i_nominal_specify=off  i_nominal_value=1  i_nominal_unit=A  v_specify=off  v_priority=None  v=0 V  v_nominal_specify=off  v_nominal_value=1  v_nominal_unit=V
  Rv : fl_lib/Electrical/Electrical Elements/Resistor  R=tb.load.R Ohm  i_specify=off  i_priority=None  i=0 A  i_nominal_specify=off  i_nominal_value=1  i_nominal_unit=A  v_specify=off  v_priority=None  v=0 V  v_nominal_specify=off  v_nominal_value=1  v_nominal_unit=V
  Rw : fl_lib/Electrical/Electrical Elements/Resistor  R=tb.load.R Ohm  i_specify=off  i_priority=None  i=0 A  i_nominal_specify=off  i_nominal_value=1  i_nominal_unit=A  v_specify=off  v_priority=None  v=0 V  v_nominal_specify=off  v_nominal_value=1  v_nominal_unit=V
  Solver Configuration : nesl_utility/Solver Configuration  PhysicalDomain=network_engine_domain  SubClassName=solver  LeftPortType=input  RightPortType=generic  Tones=[]  Harmonics=[]  SimulateNoise=off  Profile=off  UseLocalSampling=off  EnableSwitchedLinearOptims=on  FrequencyDomain=off  UseCCode=off  RelTol=0.001  AbsTol=0.001  MinStep=1e-09  ToWorkspace=off  RevertToSquareIcSolve=off  NumHomotopyIterations=100  PhasorMode=off  PhasorModeNumHarmonics=1  ConsistencySolver=NEWTON_FTOL  CanonicalOrdering=UNORDERED  OptimizeIntermediates=UNOPTIMIZED  MulticoreSolverChoice=BACKWARD_EULER  IndexReductionMethod=DerivativeReplacement  DoDC=off  ResidualTolerance=1e-4  ConsistencyTolSource=GLOBAL  ConsistencyAbsTol=0.001  ConsistencyRelTol=0.001  ConsistencyTolFactor=0.001  UseLocalSolver=on  LocalSolverChoice=NE_BACKWARD_EULER_ADVANCER  ResolveIndetEquations=on  FunctionEvalNumThread=1  LocalSolverSampleTime=tb.tc  DoFixedCost=on  MaxNonlinIter=tb.nonlin_iter_ttype  MaxModeIter=tb.mode_iter  ComputeImpulses=off  ImpulseIterations=2  LinearAlgebra=auto  LinearAlgebraNumThread=0  EquationFormulation=NE_TIME_EF  DelaysMemoryBudget=1024  AutomaticFiltering=on  FilteringTimeConstant=0.001  PartitionStorageMethod=AS_NEEDED  PartitionMemoryBudget=1024  PartitionMethod=BALANCED  MultibodyUseLocalSolver=off  MultibodyLocalSolverChoice=ODE1  MultibodyLocalSolverSampleTime=0.001
  Vdc1 : fl_lib/Electrical/Electrical Sources/DC Voltage Source  v0=tb.Vdc/2 V
  Vdc2 : fl_lib/Electrical/Electrical Sources/DC Voltage Source  v0=tb.Vdc/2 V
  i_A : nesl_utility/PS-Simulink Converter  PhysicalDomain=network_engine_domain  SubClassName=ps_output  LeftPortType=input  RightPortType=output  PseudoPeriodic=off  Frequencies=[]  VectorFormat=1-D array  Unit=A  AffineConversion=off
  i_load : fl_lib/Electrical/Electrical Sensors/Current Sensor
  three_phase_bridge_three_level_ttype_igbt_simple_2th : three_phase_bridge_three_level_ttype_igbt_simple_2th/three_phase_bridge_three_level_ttype_igbt_simple_2th  vce_sat_m=tb.igbt.vce_sat  rce_on_m=tb.igbt.rce_on  v_gamma_m=tb.igbt.v_gamma  rd_on_m=tb.igbt.rd_on  Gce_off_m=tb.igbt.Gce_off  Vth_gate_m=tb.igbt.Vth_gate  Vth_gate_hyst_m=tb.igbt.Vth_gate_hyst  Eon_m=tb.igbt.Eon  Eoff_m=tb.igbt.Eoff  Err_m=tb.igbt.Err  Ic_ref_m=tb.igbt.Ic_ref  Vdc_ref_m=tb.igbt.Vdc_ref  Vblock_Errf_m=tb.igbt.Vblock_Errf  time_constant_edge_m=tb.igbt.time_constant_edge  time_constant_ploss_m=tb.igbt.time_constant_ploss  Csnubber_m=tb.igbt.Csnubber  Rsnubber_m=tb.igbt.Rsnubber  rth_switch_JH_m=tb.igbt.rth_switch_JH  rth_switch_HA_m=tb.igbt.rth_switch_HA  rth_diode_JH_m=tb.igbt.rth_diode_JH  rth_diode_HA_m=tb.igbt.rth_diode_HA  JunctionTermalMass_m=tb.igbt.JunctionTermalMass  Tambient_m=tb.igbt.Tambient  mass_heatsink_m=tb.igbt.mass_heatsink  specific_heat_m=tb.igbt.specific_heat
  three_phase_bridge_three_level_ttype_igbt_simple_2th_i : ToWorkspace  VariableName=three_phase_bridge_three_level_ttype_igbt_simple_2th_i  SaveFormat=Timeseries  SampleTime=tb.ts_log
  three_phase_bridge_three_level_ttype_igbt_simple_2th_m : ToWorkspace  VariableName=three_phase_bridge_three_level_ttype_igbt_simple_2th_m  SaveFormat=Timeseries  SampleTime=tb.ts_log
  three_phase_bridge_three_level_ttype_igbt_simple_2th_u : ToWorkspace  VariableName=three_phase_bridge_three_level_ttype_igbt_simple_2th_u  SaveFormat=Timeseries  SampleTime=tb.ts_log
  u_V : nesl_utility/PS-Simulink Converter  PhysicalDomain=network_engine_domain  SubClassName=ps_output  LeftPortType=input  RightPortType=output  PseudoPeriodic=off  Frequencies=[]  VectorFormat=1-D array  Unit=V  AffineConversion=off
  u_load : fl_lib/Electrical/Electrical Sensors/Voltage Sensor
  wires:
  gate_commands/1 -> three_phase_bridge_three_level_ttype_igbt_simple_2th/1
  three_phase_bridge_three_level_ttype_igbt_simple_2th/1 -> three_phase_bridge_three_level_ttype_igbt_simple_2th_m/1
  i_A/1 -> three_phase_bridge_three_level_ttype_igbt_simple_2th_i/1
  u_V/1 -> three_phase_bridge_three_level_ttype_igbt_simple_2th_u/1
  connections:
  Vdc1/LConn1 -- three_phase_bridge_three_level_ttype_igbt_simple_2th/LConn1
  Vdc2/RConn1 -- three_phase_bridge_three_level_ttype_igbt_simple_2th/LConn3
  i_load/RConn1 -- i_A/LConn1
  u_load/RConn1 -- u_V/LConn1
  i_load/RConn2 -- Ru/LConn1
  Ru/RConn1 -- Lu/LConn1
  three_phase_bridge_three_level_ttype_igbt_simple_2th/RConn2 -- Rv/LConn1 -- u_load/RConn2
  Rv/RConn1 -- Lv/LConn1
  three_phase_bridge_three_level_ttype_igbt_simple_2th/RConn3 -- Rw/LConn1
  Rw/RConn1 -- Lw/LConn1
  Lu/RConn1 -- Lv/RConn1 -- Lw/RConn1
  three_phase_bridge_three_level_ttype_igbt_simple_2th/RConn1 -- i_load/LConn1 -- u_load/LConn1
  Vdc1/RConn1 -- Vdc2/LConn1 -- Electrical Reference/LConn1 -- Solver Configuration/RConn1 -- three_phase_bridge_three_level_ttype_igbt_simple_2th/LConn2

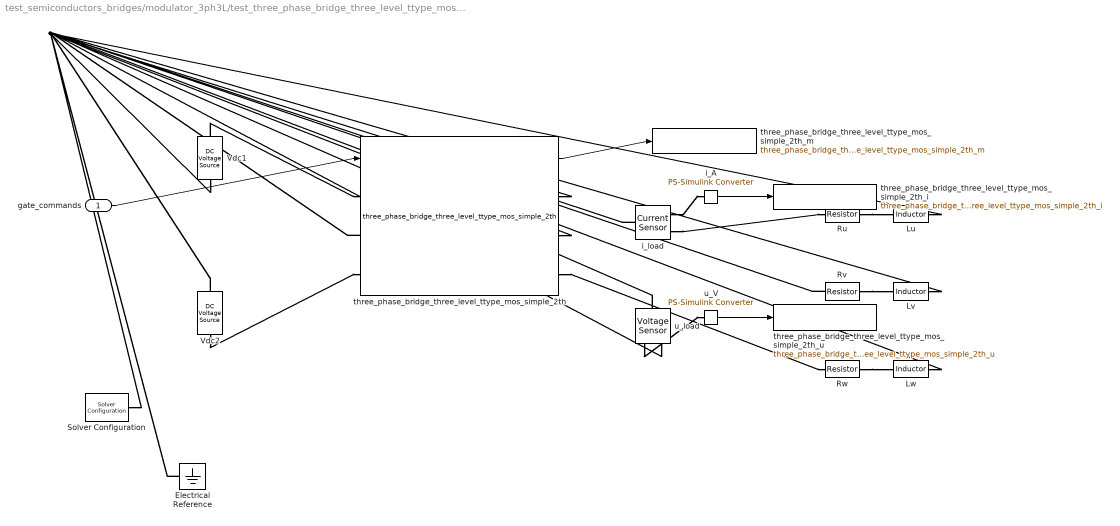
== system test_semiconductors_bridges/modulator_3ph3L/test_three_phase_bridge_three_level_ttype_mos_simple_2th ==
  gate_commands : Inport
  Electrical Reference : fl_lib/Electrical/Electrical Elements/Electrical Reference
  Lu : fl_lib/Electrical/Electrical Elements/Inductor  l=tb.load.L H  r=0 Ohm  g=0 1/Ohm  i_specify=off  i_priority=None  i=0 A  i_nominal_specify=off  i_nominal_value=1  i_nominal_unit=A  v_specify=off  v_priority=None  v=0 V  v_nominal_specify=off  v_nominal_value=1  v_nominal_unit=V  i_L_specify=off  i_L_priority=High  i_L=0 A  i_L_nominal_specify=off  i_L_nominal_value=1  i_L_nominal_unit=A
  Lv : fl_lib/Electrical/Electrical Elements/Inductor  l=tb.load.L H  r=0 Ohm  g=0 1/Ohm  i_specify=off  i_priority=None  i=0 A  i_nominal_specify=off  i_nominal_value=1  i_nominal_unit=A  v_specify=off  v_priority=None  v=0 V  v_nominal_specify=off  v_nominal_value=1  v_nominal_unit=V  i_L_specify=off  i_L_priority=High  i_L=0 A  i_L_nominal_specify=off  i_L_nominal_value=1  i_L_nominal_unit=A
  Lw : fl_lib/Electrical/Electrical Elements/Inductor  l=tb.load.L H  r=0 Ohm  g=0 1/Ohm  i_specify=off  i_priority=None  i=0 A  i_nominal_specify=off  i_nominal_value=1  i_nominal_unit=A  v_specify=off  v_priority=None  v=0 V  v_nominal_specify=off  v_nominal_value=1  v_nominal_unit=V  i_L_specify=off  i_L_priority=High  i_L=0 A  i_L_nominal_specify=off  i_L_nominal_value=1  i_L_nominal_unit=A
  Ru : fl_lib/Electrical/Electrical Elements/Resistor  R=tb.load.R Ohm  i_specify=off  i_priority=None  i=0 A  i_nominal_specify=off  i_nominal_value=1  i_nominal_unit=A  v_specify=off  v_priority=None  v=0 V  v_nominal_specify=off  v_nominal_value=1  v_nominal_unit=V
  Rv : fl_lib/Electrical/Electrical Elements/Resistor  R=tb.load.R Ohm  i_specify=off  i_priority=None  i=0 A  i_nominal_specify=off  i_nominal_value=1  i_nominal_unit=A  v_specify=off  v_priority=None  v=0 V  v_nominal_specify=off  v_nominal_value=1  v_nominal_unit=V
  Rw : fl_lib/Electrical/Electrical Elements/Resistor  R=tb.load.R Ohm  i_specify=off  i_priority=None  i=0 A  i_nominal_specify=off  i_nominal_value=1  i_nominal_unit=A  v_specify=off  v_priority=None  v=0 V  v_nominal_specify=off  v_nominal_value=1  v_nominal_unit=V
  Solver Configuration : nesl_utility/Solver Configuration  PhysicalDomain=network_engine_domain  SubClassName=solver  LeftPortType=input  RightPortType=generic  Tones=[]  Harmonics=[]  SimulateNoise=off  Profile=off  UseLocalSampling=off  EnableSwitchedLinearOptims=on  FrequencyDomain=off  UseCCode=off  RelTol=0.001  AbsTol=0.001  MinStep=1e-09  ToWorkspace=off  RevertToSquareIcSolve=off  NumHomotopyIterations=100  PhasorMode=off  PhasorModeNumHarmonics=1  ConsistencySolver=NEWTON_FTOL  CanonicalOrdering=UNORDERED  OptimizeIntermediates=UNOPTIMIZED  MulticoreSolverChoice=BACKWARD_EULER  IndexReductionMethod=DerivativeReplacement  DoDC=off  ResidualTolerance=1e-4  ConsistencyTolSource=GLOBAL  ConsistencyAbsTol=0.001  ConsistencyRelTol=0.001  ConsistencyTolFactor=0.001  UseLocalSolver=on  LocalSolverChoice=NE_BACKWARD_EULER_ADVANCER  ResolveIndetEquations=on  FunctionEvalNumThread=1  LocalSolverSampleTime=tb.tc  DoFixedCost=on  MaxNonlinIter=tb.nonlin_iter_ttype  MaxModeIter=tb.mode_iter  ComputeImpulses=off  ImpulseIterations=2  LinearAlgebra=auto  LinearAlgebraNumThread=0  EquationFormulation=NE_TIME_EF  DelaysMemoryBudget=1024  AutomaticFiltering=on  FilteringTimeConstant=0.001  PartitionStorageMethod=AS_NEEDED  PartitionMemoryBudget=1024  PartitionMethod=BALANCED  MultibodyUseLocalSolver=off  MultibodyLocalSolverChoice=ODE1  MultibodyLocalSolverSampleTime=0.001
  Vdc1 : fl_lib/Electrical/Electrical Sources/DC Voltage Source  v0=tb.Vdc/2 V
  Vdc2 : fl_lib/Electrical/Electrical Sources/DC Voltage Source  v0=tb.Vdc/2 V
  i_A : nesl_utility/PS-Simulink Converter  PhysicalDomain=network_engine_domain  SubClassName=ps_output  LeftPortType=input  RightPortType=output  PseudoPeriodic=off  Frequencies=[]  VectorFormat=1-D array  Unit=A  AffineConversion=off
  i_load : fl_lib/Electrical/Electrical Sensors/Current Sensor
  three_phase_bridge_three_level_ttype_mos_simple_2th : three_phase_bridge_three_level_ttype_mos_simple_2th/three_phase_bridge_three_level_ttype_mos_simple_2th  rds_on_m=tb.mos.rds_on  alpha_R_m=tb.mos.alpha_R  Tj_ref_m=tb.mos.Tj_ref  Roff_m=tb.mos.Roff  v_gamma_m=tb.mos.v_gamma  rd_on_m=tb.mos.rd_on  two_die_m=tb.mos.two_die  G_th_m=tb.mos.G_th  Eon_m=tb.mos.Eon  Eoff_m=tb.mos.Eoff  Err_m=tb.mos.Err  Ic_ref_m=tb.mos.Ic_ref  Vdc_ref_m=tb.mos.Vdc_ref  ki_m=tb.mos.ki  kv_m=tb.mos.kv  Vth_off_m=tb.mos.Vth_off  Vth_on_m=tb.mos.Vth_on  V_sm_m=tb.mos.V_sm  time_constant_edge_m=tb.mos.time_constant_edge  tau_v_m=tb.mos.tau_v  time_constant_ploss_m=tb.mos.time_constant_ploss  i_eps_m=tb.mos.i_eps  Csnubber_m=tb.mos.Csnubber  Rsnubber_m=tb.mos.Rsnubber  rth_switch_JH_m=tb.mos.rth_switch_JH  rth_switch_HA_m=tb.mos.rth_switch_HA  rth_diode_JH_m=tb.mos.rth_diode_JH  rth_diode_HA_m=tb.mos.rth_diode_HA  JunctionTermalMass_m=tb.mos.JunctionTermalMass  Tambient_m=tb.mos.Tambient  mass_heatsink_m=tb.mos.mass_heatsink  specific_heat_m=tb.mos.specific_heat
  three_phase_bridge_three_level_ttype_mos_simple_2th_i : ToWorkspace  VariableName=three_phase_bridge_three_level_ttype_mos_simple_2th_i  SaveFormat=Timeseries  SampleTime=tb.ts_log
  three_phase_bridge_three_level_ttype_mos_simple_2th_m : ToWorkspace  VariableName=three_phase_bridge_three_level_ttype_mos_simple_2th_m  SaveFormat=Timeseries  SampleTime=tb.ts_log
  three_phase_bridge_three_level_ttype_mos_simple_2th_u : ToWorkspace  VariableName=three_phase_bridge_three_level_ttype_mos_simple_2th_u  SaveFormat=Timeseries  SampleTime=tb.ts_log
  u_V : nesl_utility/PS-Simulink Converter  PhysicalDomain=network_engine_domain  SubClassName=ps_output  LeftPortType=input  RightPortType=output  PseudoPeriodic=off  Frequencies=[]  VectorFormat=1-D array  Unit=V  AffineConversion=off
  u_load : fl_lib/Electrical/Electrical Sensors/Voltage Sensor
  wires:
  gate_commands/1 -> three_phase_bridge_three_level_ttype_mos_simple_2th/1
  three_phase_bridge_three_level_ttype_mos_simple_2th/1 -> three_phase_bridge_three_level_ttype_mos_simple_2th_m/1
  i_A/1 -> three_phase_bridge_three_level_ttype_mos_simple_2th_i/1
  u_V/1 -> three_phase_bridge_three_level_ttype_mos_simple_2th_u/1
  connections:
  Vdc1/LConn1 -- three_phase_bridge_three_level_ttype_mos_simple_2th/LConn1
  Vdc2/RConn1 -- three_phase_bridge_three_level_ttype_mos_simple_2th/LConn3
  i_load/RConn1 -- i_A/LConn1
  u_load/RConn1 -- u_V/LConn1
  i_load/RConn2 -- Ru/LConn1
  Ru/RConn1 -- Lu/LConn1
  three_phase_bridge_three_level_ttype_mos_simple_2th/RConn2 -- Rv/LConn1 -- u_load/RConn2
  Rv/RConn1 -- Lv/LConn1
  three_phase_bridge_three_level_ttype_mos_simple_2th/RConn3 -- Rw/LConn1
  Rw/RConn1 -- Lw/LConn1
  Lu/RConn1 -- Lv/RConn1 -- Lw/RConn1
  three_phase_bridge_three_level_ttype_mos_simple_2th/RConn1 -- i_load/LConn1 -- u_load/LConn1
  Vdc1/RConn1 -- Vdc2/LConn1 -- Electrical Reference/LConn1 -- Solver Configuration/RConn1 -- three_phase_bridge_three_level_ttype_mos_simple_2th/LConn2
